simulink model "FW_SkySurfer_HIL"  (R2026b)
settings: Solver=ode4  StopTime=inf  FixedStep=Thil  EnableMultiTasking=on
PreLoadFcn:
  | % Load this folder's HIL settings and MAVLink Bus types (not another project's).
  | run(fullfile(fileparts(get_param(bdroot,'FileName')),'PX4_HIL_preload.m'));
InitFcn:
  | % Record the model first: loading libraries can change the current diagram.
  | assignin('base','lastRunModel',bdroot);
  | % Rebuild HIL settings/Bus types (also after clear all), then aircraft data.
  | hilModelFolder = fileparts(get_param(lastRunModel,'FileName'));
  | run(fullfile(hilModelFolder,'PX4_HIL_preload.m'));
  | run(fullfile(hilModelFolder,'FW_SkySurfer_InitialFunction.m'));
  | clear hilModelFolder
values from neighbouring files (symbols this model uses):
  Aeroelasticity_AIL = [   5   15]    [FW_SkySurfer_InitialFunction.m]
  Aeroelasticity_ELE = [   5   15]    [FW_SkySurfer_InitialFunction.m]
  Aeroelasticity_Gain_AIL = [ 0.8  0.5]    [FW_SkySurfer_InitialFunction.m]
  Aeroelasticity_Gain_ELE = [ 0.9  0.6]    [FW_SkySurfer_InitialFunction.m]
  Aeroelasticity_Gain_RUD = [ 0.9  0.6]    [FW_SkySurfer_InitialFunction.m]
  Aeroelasticity_RUD = [   5   15]    [FW_SkySurfer_InitialFunction.m]
  alpha_avl = [-10 -5 0 5 10 15]    [import_aerostates_avl.m]
  AoA = [-10 -5 0 5 10 15]    [import_aerostates_vsp.m]
  AoS = [-10 0 10]    [import_aerostates_vsp.m]
  b = 1.41    [FW_SkySurfer_InitialFunction.m]
  beta_avl = [-10 -5 0 5 10]    [import_aerostates_avl.m]
  C_wgrp = struct()    [import_aerostates_vsp.m]
  cbar = 0.20    (= 0.2)    [FW_SkySurfer_InitialFunction.m]
  CD_fix_AVL = 0.075    [FW_SkySurfer_InitialFunction.m]
  CD_fix_VSP = 0.065    [FW_SkySurfer_InitialFunction.m]
  CDd01 = zeros(length(mach_avl), length(alpha_avl), length(beta_avl))    [import_aerostates_avl.m]
  CDd02 = zeros(length(mach_avl), length(alpha_avl), length(beta_avl))    [import_aerostates_avl.m]
  CDd03 = zeros(length(mach_avl), length(alpha_avl), length(beta_avl))    [import_aerostates_avl.m]
  CDd04 = zeros(length(mach_avl), length(alpha_avl), length(beta_avl))    [import_aerostates_avl.m]
  CDp = zeros(length(mach_avl), length(alpha_avl), length(beta_avl))    [import_aerostates_avl.m]
  CDq = zeros(length(mach_avl), length(alpha_avl), length(beta_avl))    [import_aerostates_avl.m]
  CDr = zeros(length(mach_avl), length(alpha_avl), length(beta_avl))    [import_aerostates_avl.m]
  CDtot = zeros(length(mach_avl), length(alpha_avl), length(beta_avl))    [import_aerostates_avl.m]
  CG_m = [0.330, 0, 0]    [FW_SkySurfer_InitialFunction.m]
  CLd01 = zeros(length(mach_avl), length(alpha_avl), length(beta_avl))    [import_aerostates_avl.m]
  Cld01 = zeros(length(mach_avl), length(alpha_avl), length(beta_avl))    [import_aerostates_avl.m]
  CLd02 = zeros(length(mach_avl), length(alpha_avl), length(beta_avl))    [import_aerostates_avl.m]
  Cld02 = zeros(length(mach_avl), length(alpha_avl), length(beta_avl))    [import_aerostates_avl.m]
  CLd03 = zeros(length(mach_avl), length(alpha_avl), length(beta_avl))    [import_aerostates_avl.m]
  Cld03 = zeros(length(mach_avl), length(alpha_avl), length(beta_avl))    [import_aerostates_avl.m]
  CLd04 = zeros(length(mach_avl), length(alpha_avl), length(beta_avl))    [import_aerostates_avl.m]
  Cld04 = zeros(length(mach_avl), length(alpha_avl), length(beta_avl))    [import_aerostates_avl.m]
  CLp = zeros(length(mach_avl), length(alpha_avl), length(beta_avl))    [import_aerostates_avl.m]
  Clp = zeros(length(mach_avl), length(alpha_avl), length(beta_avl))    [import_aerostates_avl.m]
  CLq = zeros(length(mach_avl), length(alpha_avl), length(beta_avl))    [import_aerostates_avl.m]
  Clq = zeros(length(mach_avl), length(alpha_avl), length(beta_avl))    [import_aerostates_avl.m]
  CLr = zeros(length(mach_avl), length(alpha_avl), length(beta_avl))    [import_aerostates_avl.m]
  Clr = zeros(length(mach_avl), length(alpha_avl), length(beta_avl))    [import_aerostates_avl.m]
  CLtot = zeros(length(mach_avl), length(alpha_avl), length(beta_avl))    [import_aerostates_avl.m]
  Cltot = zeros(length(mach_avl), length(alpha_avl), length(beta_avl))    [import_aerostates_avl.m]
  Cmd01 = zeros(length(mach_avl), length(alpha_avl), length(beta_avl))    [import_aerostates_avl.m]
  Cmd02 = zeros(length(mach_avl), length(alpha_avl), length(beta_avl))    [import_aerostates_avl.m]
  Cmd03 = zeros(length(mach_avl), length(alpha_avl), length(beta_avl))    [import_aerostates_avl.m]
  Cmd04 = zeros(length(mach_avl), length(alpha_avl), length(beta_avl))    [import_aerostates_avl.m]
  Cmp = zeros(length(mach_avl), length(alpha_avl), length(beta_avl))    [import_aerostates_avl.m]
  Cmq = zeros(length(mach_avl), length(alpha_avl), length(beta_avl))    [import_aerostates_avl.m]
  Cmr = zeros(length(mach_avl), length(alpha_avl), length(beta_avl))    [import_aerostates_avl.m]
  Cmtot = zeros(length(mach_avl), length(alpha_avl), length(beta_avl))    [import_aerostates_avl.m]
  Cnd01 = zeros(length(mach_avl), length(alpha_avl), length(beta_avl))    [import_aerostates_avl.m]
  Cnd02 = zeros(length(mach_avl), length(alpha_avl), length(beta_avl))    [import_aerostates_avl.m]
  Cnd03 = zeros(length(mach_avl), length(alpha_avl), length(beta_avl))    [import_aerostates_avl.m]
  Cnd04 = zeros(length(mach_avl), length(alpha_avl), length(beta_avl))    [import_aerostates_avl.m]
  Cnp = zeros(length(mach_avl), length(alpha_avl), length(beta_avl))    [import_aerostates_avl.m]
  Cnq = zeros(length(mach_avl), length(alpha_avl), length(beta_avl))    [import_aerostates_avl.m]
  Cnr = zeros(length(mach_avl), length(alpha_avl), length(beta_avl))    [import_aerostates_avl.m]
  Cntot = zeros(length(mach_avl), length(alpha_avl), length(beta_avl))    [import_aerostates_avl.m]
  CYd01 = zeros(length(mach_avl), length(alpha_avl), length(beta_avl))    [import_aerostates_avl.m]
  CYd02 = zeros(length(mach_avl), length(alpha_avl), length(beta_avl))    [import_aerostates_avl.m]
  CYd03 = zeros(length(mach_avl), length(alpha_avl), length(beta_avl))    [import_aerostates_avl.m]
  CYd04 = zeros(length(mach_avl), length(alpha_avl), length(beta_avl))    [import_aerostates_avl.m]
  CYp = zeros(length(mach_avl), length(alpha_avl), length(beta_avl))    [import_aerostates_avl.m]
  CYq = zeros(length(mach_avl), length(alpha_avl), length(beta_avl))    [import_aerostates_avl.m]
  CYr = zeros(length(mach_avl), length(alpha_avl), length(beta_avl))    [import_aerostates_avl.m]
  CYtot = zeros(length(mach_avl), length(alpha_avl), length(beta_avl))    [import_aerostates_avl.m]
  del_z = 0    [FW_SkySurfer_InitialFunction.m]
  g = 9.80665    [FW_SkySurfer_InitialFunction.m]
  H0 = 1000 * convlength(1, 'ft', 'm')    [FW_SkySurfer_InitialFunction.m]
  Inertia0 = [  Ixx -Ixy -Ixz  ;                              -Ixy  Iyy -Iyz  ;                              -Ixz -Iyz  Izz ]    [FW_SkySurfer_InitialFunction.m]
  Lat0 = 22.910275834988674    (= 22.910275835)    [FW_SkySurfer_InitialFunction.m]
  Lon0 = 120.31096929726908    (= 120.310969297)    [FW_SkySurfer_InitialFunction.m]
  Mach = [0.05 0.10]    [import_aerostates_vsp.m]
  mach_avl = [0.05 0.10]    [import_aerostates_avl.m]
  Mass0 = 1.3    [FW_SkySurfer_InitialFunction.m]
  Phi0 = 0    [FW_SkySurfer_InitialFunction.m]
  Psi0 = 0    [FW_SkySurfer_InitialFunction.m]
  Psi_w = 0    [FW_SkySurfer_InitialFunction.m]
  Theta0 = 0.8633    [FW_SkySurfer_InitialFunction.m]
  Thil = 1/250    (= 0.004)    [FW_SkySurfer_InitialFunction.m]
  U0 = 40.0309 * convvel(1, 'kts', 'm/s')    [FW_SkySurfer_InitialFunction.m]
  useAVL_VSP = 0    [FW_SkySurfer_InitialFunction.m]
  V0 = 0    [FW_SkySurfer_InitialFunction.m]
  Vel_w = 0    [FW_SkySurfer_InitialFunction.m]
  W0 = 0.6032 * convvel(1, 'kts', 'm/s')    [FW_SkySurfer_InitialFunction.m]
  XREF_m = [0.330, 0, 0]    [FW_SkySurfer_InitialFunction.m]
undefined symbols (not defined in the file or in its folder): F, Light, m, MIL, Newton, Raphson, s, Ts, uavData
libraries: simulink_extras x28, aerolibasang x5, shared6dofsys x4, aerolibwind2 x4, sharedtransform x3, sharedutil x2, shared6dof x2, simulink x1, aerolibatmos2 x1, aerolibconvert2 x1
(part 3 of 3)

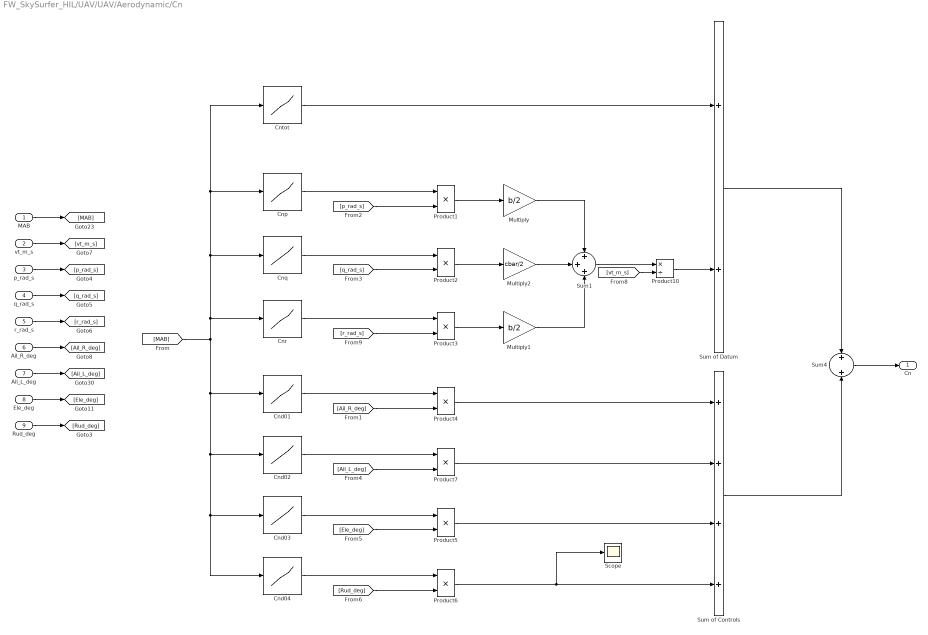
== system FW_SkySurfer_HIL/UAV/UAV/Aerodynamic/Cn ==
  MAB : Inport
  vt_m_s : Inport  Port=2
  p_rad_s : Inport  Port=3
  q_rad_s : Inport  Port=4
  r_rad_s : Inport  Port=5
  Ail_R_deg : Inport  Port=6
  Ail_L_deg : Inport  Port=7
  Ele_deg : Inport  Port=8
  Rud_deg : Inport  Port=9
  Cnd01 : Lookup_n-D  NumberOfTableDimensions=3  BreakpointsForDimension1=mach_avl  BreakpointsForDimension2=alpha_avl  BreakpointsForDimension3=beta_avl  UseOneInputPortForAllInputData=on  Table=Cnd01  InternalRulePriority=Speed  RndMeth=Simplest
  Cnd02 : Lookup_n-D  NumberOfTableDimensions=3  BreakpointsForDimension1=mach_avl  BreakpointsForDimension2=alpha_avl  BreakpointsForDimension3=beta_avl  UseOneInputPortForAllInputData=on  Table=Cnd02  InternalRulePriority=Speed  RndMeth=Simplest
  Cnd03 : Lookup_n-D  NumberOfTableDimensions=3  BreakpointsForDimension1=mach_avl  BreakpointsForDimension2=alpha_avl  BreakpointsForDimension3=beta_avl  UseOneInputPortForAllInputData=on  Table=Cnd03  InternalRulePriority=Speed  RndMeth=Simplest
  Cnd04 : Lookup_n-D  NumberOfTableDimensions=3  BreakpointsForDimension1=mach_avl  BreakpointsForDimension2=alpha_avl  BreakpointsForDimension3=beta_avl  UseOneInputPortForAllInputData=on  Table=Cnd04  InternalRulePriority=Speed  RndMeth=Simplest
  Cnp : Lookup_n-D  NumberOfTableDimensions=3  BreakpointsForDimension1=mach_avl  BreakpointsForDimension2=alpha_avl  BreakpointsForDimension3=beta_avl  UseOneInputPortForAllInputData=on  Table=Cnp  InternalRulePriority=Speed  RndMeth=Simplest
  Cnq : Lookup_n-D  NumberOfTableDimensions=3  BreakpointsForDimension1=mach_avl  BreakpointsForDimension2=alpha_avl  BreakpointsForDimension3=beta_avl  UseOneInputPortForAllInputData=on  Table=Cnq  InternalRulePriority=Speed  RndMeth=Simplest
  Cnr : Lookup_n-D  NumberOfTableDimensions=3  BreakpointsForDimension1=mach_avl  BreakpointsForDimension2=alpha_avl  BreakpointsForDimension3=beta_avl  UseOneInputPortForAllInputData=on  Table=Cnr  InternalRulePriority=Speed  RndMeth=Simplest
  Cntot : Lookup_n-D  NumberOfTableDimensions=3  BreakpointsForDimension1=mach_avl  BreakpointsForDimension2=alpha_avl  BreakpointsForDimension3=beta_avl  UseOneInputPortForAllInputData=on  Table=Cntot  InternalRulePriority=Speed  RndMeth=Simplest
  Multiply : Gain  Gain=b/2
  Multiply1 : Gain  Gain=b/2
  Multiply2 : Gain  Gain=cbar/2
  Product{1..7} (7 alike) : Product
  Product10 : Product  Inputs=*/  InputSameDT=on  SaturateOnIntegerOverflow=on  OutDataTypeStr=Inherit: Same as first input
  Scope : Scope
      settings: ActiveDisplayYMinimum=-1  ActiveDisplayYMaximum=1  DataLoggingVariableName=ScopeData25
  Sum of Controls : Sum  Inputs=++++
  Sum of Datum : Sum
  Sum1 : Sum  Inputs=+++  InputSameDT=on  SaturateOnIntegerOverflow=on  OutDataTypeStr=Inherit: Same as first input
  Sum4 : Sum  InputSameDT=on  SaturateOnIntegerOverflow=on  OutDataTypeStr=Inherit: Same as first input
  Cn : Outport
  wires:
  q_rad_s/1 -> [q_rad_s]
  vt_m_s/1 -> [vt_m_s]
  p_rad_s/1 -> [p_rad_s]
  Ail_L_deg/1 -> [Ail_L_deg]
  Ail_R_deg/1 -> [Ail_R_deg]
  MAB/1 -> [MAB]
  r_rad_s/1 -> [r_rad_s]
  Rud_deg/1 -> [Rud_deg]
  Ele_deg/1 -> [Ele_deg]
  Cnp/1 -> Product1/1
  Cnd03/1 -> Product5/1
  Cnd04/1 -> Product6/1
  [Ail_L_deg] -> Product7/2
  Product3/1 -> Multiply1/1
  Product5/1 -> Sum of Controls/3
  Cnr/1 -> Product3/1
  Multiply/1 -> Sum1/1
  Product6/1 -> Scope/1, Sum of Controls/4
  Cnd02/1 -> Product7/1
  [Rud_deg] -> Product6/2
  Product10/1 -> Sum of Datum/2
  Multiply2/1 -> Sum1/2
  Sum of Controls/1 -> Sum4/2
  Product7/1 -> Sum of Controls/2
  Product2/1 -> Multiply2/1
  [Ele_deg] -> Product5/2
  [q_rad_s] -> Product2/2
  Sum1/1 -> Product10/1
  Product4/1 -> Sum of Controls/1
  [p_rad_s] -> Product1/2
  [Ail_R_deg] -> Product4/2
  [MAB] -> Cnr/1, Cnq/1, Cnp/1, Cntot/1, Cnd01/1, Cnd02/1, Cnd04/1, Cnd03/1
  Cntot/1 -> Sum of Datum/1
  [r_rad_s] -> Product3/2
  Cnq/1 -> Product2/1
  Cnd01/1 -> Product4/1
  Sum4/1 -> Cn/1
  Multiply1/1 -> Sum1/3
  Sum of Datum/1 -> Sum4/1
  [vt_m_s] -> Product10/2
  Product1/1 -> Multiply/1

== system FW_SkySurfer_HIL/UAV/UAV/Environment/Gravity ==
  DCM : Inport
  Constant : Constant  Value=[0; 0; g]  VectorParams1D=off
  Product : Product  Multiplication=Matrix(*)  InputSameDT=on  RndMeth=Zero  SaturateOnIntegerOverflow=on  OutDataTypeStr=Inherit: Same as first input
  Product3 : Product  RndMeth=Zero
  Gravity : Outport
  wires:
  Product/1 -> Product3/2
  Product3/1 -> Gravity/1
  Constant/1 -> Product/2
  DCM/1 -> Product/1
  [mass] -> Product3/1

== system FW_SkySurfer_HIL/UAV/UAV/Environment/Wind ==
  note: WIND_IDX = 2
  note: WIND_IDX = 1
  WIND_IDX : Inport
  wind.Vel : Inport  Port=2
  wind.Psi : Inport  Port=3
  AR : MultiPortSwitch  Inputs=2  SaturateOnIntegerOverflow=off  InputSameDT=off
  Constant2 : Constant  Value=[0; 0; 0]  VectorParams1D=off  SampleTime=-1
  Discrete Wind Gust Model - On : aerolibwind2/Discrete Wind Gust Model  units=Metric (MKS)  Gx=on  Gy=on  Gz=on  t_0=20  d_m=[120 120 80]  v_m=[3.5 3.0 3.0]
  Dryden Wind Turbulence Model (Continuous (+q -r)) : aerolibwind2/Dryden Wind Turbulence Model  (Continuous (+q -r))  units=Metric (MKS)  spec=MIL-F-8785C  model=Continuous Dryden (+q -r)  W20=0  Wdeg=0  TurbProb=10^-2 - Light  L_high=533.4  Wingspan=4  ts=Thil  Seed=[23341 23342 23343 23344]  T_on=on
  Dryden airspeed floor : Saturate  Description=Dryden divides by airspeed: below the 5 m/s aero cut-in the turbulence filters use 5 m/s (0 m/s on the ground made the derivatives infinite; why the block had been commented out).  UpperLimit=inf  LowerLimit=5
  Horizontal Wind Model : aerolibwind2/Horizontal Wind Model  units=Metric (MKS)  Vw_source=External  Vwind=15  W_source=External  Wdeg=0
  Sum : Sum  Inputs=+++  InputSameDT=on  SaturateOnIntegerOverflow=on  OutDataTypeStr=Inherit: Same as first input
  VB : MultiPortSwitch  Inputs=2  SaturateOnIntegerOverflow=off  InputSameDT=off
  Velocity Conversion3 : aerolibconvert2/Velocity Conversion  IU=kts  OU=m/s
  Wind Shear Model : aerolibwind2/Wind Shear Model  units=Metric (MKS)  phase=Category C - Terminal Flight Phase  W_20=0  Wdeg=0
  wind.UVW : Outport
  wind.PQR : Outport  Port=2
  wires:
  WIND_IDX/1 -> VB/1, AR/1
  AR/1 -> wind.PQR/1
  VB/1 -> wind.UVW/1
  [wAR2] -> AR/3
  [wVB] -> VB/2
  Horizontal Wind Model/1 -> [wVB]
  [wVB2] -> VB/3
  wind.Vel/1 -> Velocity Conversion3/1
  Velocity Conversion3/1 -> Horizontal Wind Model/2
  wind.Psi/1 -> Horizontal Wind Model/3
  [DCM] -> Wind Shear Model/2, Dryden Wind Turbulence Model (Continuous (+q -r))/3
  Wind Shear Model/1 -> Sum/2
  [H] -> Wind Shear Model/1, Dryden Wind Turbulence Model (Continuous (+q -r))/1
  Discrete Wind Gust Model - On/1 -> Sum/1
  Dryden Wind Turbulence Model (Continuous (+q -r))/1 -> Sum/3
  Dryden Wind Turbulence Model (Continuous (+q -r))/2 -> [wAR2]
  Sum/1 -> [wVB2]
  [U] -> Discrete Wind Gust Model - On/1, Dryden airspeed floor/1
  [DCM] -> Horizontal Wind Model/1
  Constant2/1 -> AR/2
  Dryden airspeed floor/1 -> Dryden Wind Turbulence Model (Continuous (+q -r))/2

== system FW_SkySurfer_HIL/UAV/UAV/Ground Model/Friction Force ==
  V : Inport
  Fn : Inport  Port=2
  Product : Product
  Soft Coulomb Friction : Subsystem
  Unary Minus : UnaryMinus
  Friction : Outport
  wires:
  Fn/1 -> Product/2
  Soft Coulomb Friction/1(Out1) -> Product/1
  Product/1 -> Unary Minus/1
  Unary Minus/1 -> Friction/1
  V/1 -> Soft Coulomb Friction/1(V)

== system FW_SkySurfer_HIL/UAV/UAV/Ground Model/Normal Force ==
  Vz : Inport
  Z : Inport  Port=2
  Add : Sum
  Constant : Constant  Value=0
  Damper : Gain  Gain=-uavData.contact.damper
  Saturation : Saturate  UpperLimit=inf  LowerLimit=0
  Spring Kp : Gain  Gain=-uavData.contact.spring
  Switch : Switch  Criteria=u2 > Threshold  SaturateOnIntegerOverflow=off  InputSameDT=off
  Unary Minus : UnaryMinus
  Unary Minus1 : UnaryMinus
  Normal : Outport
  wires:
  Constant/1 -> Switch/1
  Z/1 -> Unary Minus/1
  Switch/1 -> Saturation/1
  Damper/1 -> Add/2
  Add/1 -> Switch/3
  Spring Kp/1 -> Add/1
  Vz/1 -> Unary Minus1/1
  Saturation/1 -> Normal/1
  Unary Minus/1 -> Spring Kp/1, Switch/2
  Unary Minus1/1 -> Damper/1

== system FW_SkySurfer_HIL/UAV/UAV/Measurement/Subsystem ==
  Vb : Inport
  Airspeed : Sqrt  RsqrtAlgorithmType=Newton-Raphson
  Constant2 : Constant  Value=0  VectorParams1D=off
  Incidence : Trigonometry  Operator=atan2
  Product : Product  Inputs=*/  SaturateOnIntegerOverflow=on  OutDataTypeStr=Inherit: Same as first input
  Sideslip : Trigonometry  Operator=asin
  Subsystem : aerolibasang/Incidence, Sideslip, & Airspeed/Subsystem  SystemSampleTime=-1  VariantActivationTime=update diagram  EmptyChoice=off  PassThrough=off  PassThroughVariantControl=(default)  EmptyChoiceVariantControl=(default)  AllowFlexibleInterface=on  Latency=0  AutoFrameSizeCalculation=off
  Subsystem1 : aerolibasang/Incidence, Sideslip, & Airspeed/Subsystem1  SystemSampleTime=-1  VariantActivationTime=update diagram  EmptyChoice=off  PassThrough=off  PassThroughVariantControl=(default)  EmptyChoiceVariantControl=(default)  AllowFlexibleInterface=on  Latency=0  AutoFrameSizeCalculation=off
  Switch : Switch  Criteria=u2 > Threshold  SaturateOnIntegerOverflow=off  InputSameDT=off
  dot : aerolibasang/Incidence, Sideslip, & Airspeed/dot  SystemSampleTime=-1  VariantActivationTime=update diagram  EmptyChoice=off  PassThrough=off  PassThroughVariantControl=(default)  EmptyChoiceVariantControl=(default)  AllowFlexibleInterface=on  Latency=0  AutoFrameSizeCalculation=off
  Alpha : Outport  Unit=rad  InitialOutput=0  VectorParamsAs1DForOutWhenUnconnected=off
  Beta : Outport  Port=2  Unit=rad  InitialOutput=0  VectorParamsAs1DForOutWhenUnconnected=off
  V : Outport  Port=3  InitialOutput=0  VectorParamsAs1DForOutWhenUnconnected=off
  wires:
  Subsystem1/1 -> Product/1
  Airspeed/1 -> V/1, Product/2, Switch/2
  Vb/1 -> Subsystem/1, Subsystem1/1, dot/1
  Product/1 -> Sideslip/1
  dot/1 -> Airspeed/1
  Subsystem/2 -> Incidence/2
  Subsystem/1 -> Incidence/1
  Sideslip/1 -> Switch/1
  Constant2/1 -> Switch/3
  Incidence/1 -> Alpha/1
  Switch/1 -> Beta/1

== system FW_SkySurfer_HIL/UAV/UAV/Ground Model/Friction Force/Soft Coulomb Friction ==
  note: Pennestrì, E., Rossi, V., Salvini, P. et al. Review and comparison of dry friction force models. Nonlinear Dyn 83, 1785–1801 (2016). https://doi.org/10.1007/s11071-015-2485-3
  V : Inport
  Tanh : Trigonometry  Operator=tanh
  friction coefficient : Gain  Gain=uavData.contact.rollingFriction
  vd : Gain  Gain=1/uavData.contact.vd
  Out1 : Outport
  wires:
  V/1 -> vd/1
  vd/1 -> Tanh/1
  Tanh/1 -> friction coefficient/1
  friction coefficient/1 -> Out1/1
